simulink model "physical_lab5_bandwidth"  (R2024b)
settings: Solver=ode15s  StartTime=0.0  StopTime=0.0001  MaxStep=1.6666666666666667e-08  RelTol=1e-7  AbsTol=1e-9
model workspace (MAT data in the model file):
  physical_input = timeseries
  physical_input.Name = 'unnamed'
  physical_input.DataInfo = tsdata.datametadata
  physical_input.DataInfo.Interpolation = tsdata.interpolation
  physical_input.DataInfo.Interpolation.Fhandle : function handle (value not decoded)
  physical_input.DataInfo.Interpolation.Name = 'linear'
  physical_input.TimeInfo = tsdata.timemetadata
  physical_input.TimeInfo.Length = 6001
  physical_input.TimeInfo.DuplicateTimes = 0
  physical_input.TimeInfo.Time_ = [0 1.66666666667e-08 3.33333333333e-08 5e-08 6.66666666667e-08 8.33333333333e-08 1e-07 1.16666666667e-07 1.33333333333e-07 1.5e-07 1.66666666667e-07 1.83333333333e-07 ... (6001 elements, 6001x1)]
  physical_input.TimeInfo.Initialized = 1
  physical_input.QualityInfo = tsdata.qualmetadata
  physical_input.Data_ = [0 0.000523589205812 0.00104712099417 0.00157053795391 0.00209378268646 0.00261679781215 0.00313952597647 0.00366190985638 0.00418389216662 0.00470541566593 0.00522642316338 0.00574685752464 ... (6001 elements, 6001x1)]
libraries: fl_lib x13, nesl_utility x7
settings Model: Creator=33657  LastModifiedBy=33657

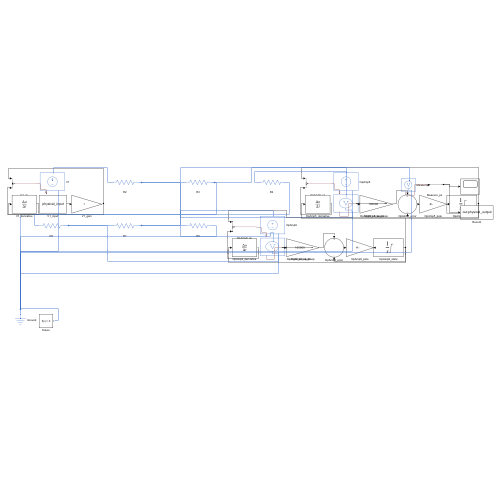
[thumbnail: Simulink's stored preview of the top-level diagram]
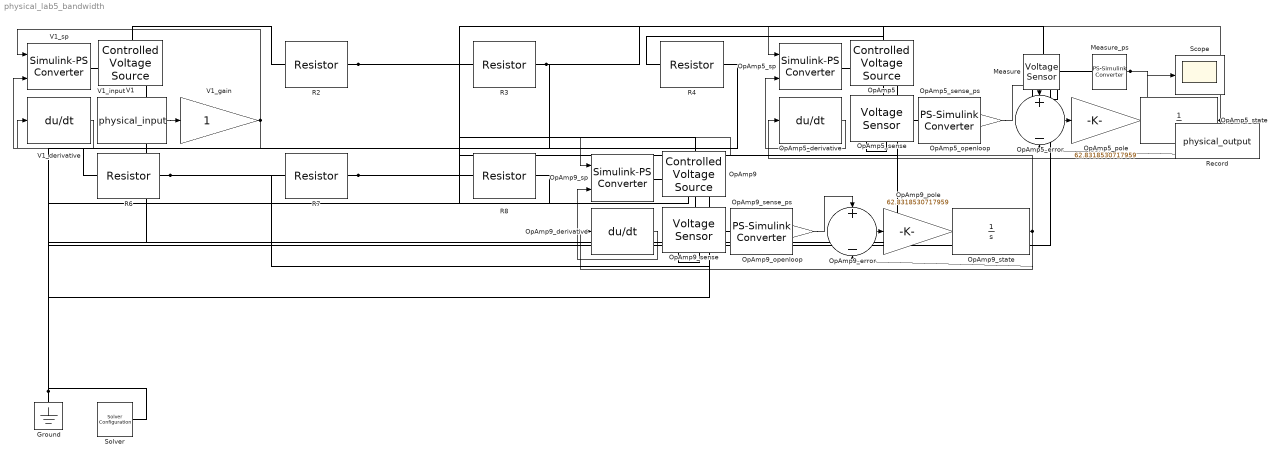
== system physical_lab5_bandwidth ==
  Ground : fl_lib/Electrical/Electrical Elements/Electrical Reference
  Measure : fl_lib/Electrical/Electrical Sensors/Voltage Sensor
  Measure_ps : nesl_utility/PS-Simulink Converter  PhysicalDomain=network_engine_domain  SubClassName=ps_output  LeftPortType=input  RightPortType=output  PseudoPeriodic=off  Frequencies=[]  VectorFormat=inherit  Unit=V  AffineConversion=off
  OpAmp5 : fl_lib/Electrical/Electrical Sources/Controlled Voltage Source
  OpAmp5_derivative : Derivative
  OpAmp5_error : Sum  Inputs=+-
  OpAmp5_openloop : Gain  Gain=100000
  OpAmp5_pole : Gain  Gain=62.8318530717959
  OpAmp5_sense : fl_lib/Electrical/Electrical Sensors/Voltage Sensor
  OpAmp5_sense_ps : nesl_utility/PS-Simulink Converter  PhysicalDomain=network_engine_domain  SubClassName=ps_output  LeftPortType=input  RightPortType=output  PseudoPeriodic=off  Frequencies=[]  VectorFormat=inherit  Unit=V  AffineConversion=off
  OpAmp5_sp : nesl_utility/Simulink-PS Converter  PhysicalDomain=network_engine_domain  SubClassName=ps_input  LeftPortType=input  RightPortType=output  PseudoPeriodic=off  Frequencies=[]  NoiseDistribution=none  NoiseParameters=[]  Unit=V  AffineConversion=off  FilteringAndDerivatives=provide  SimscapeFilterOrder=1  InputFilterTimeConstant=0.001  UdotUserProvided=1
  OpAmp5_state : Integrator  LimitOutput=on  UpperSaturationLimit=15  LowerSaturationLimit=-15
  OpAmp9 : fl_lib/Electrical/Electrical Sources/Controlled Voltage Source
  OpAmp9_derivative : Derivative
  OpAmp9_error : Sum  Inputs=+-
  OpAmp9_openloop : Gain  Gain=100000
  OpAmp9_pole : Gain  Gain=62.8318530717959
  OpAmp9_sense : fl_lib/Electrical/Electrical Sensors/Voltage Sensor
  OpAmp9_sense_ps : nesl_utility/PS-Simulink Converter  PhysicalDomain=network_engine_domain  SubClassName=ps_output  LeftPortType=input  RightPortType=output  PseudoPeriodic=off  Frequencies=[]  VectorFormat=inherit  Unit=V  AffineConversion=off
  OpAmp9_sp : nesl_utility/Simulink-PS Converter  PhysicalDomain=network_engine_domain  SubClassName=ps_input  LeftPortType=input  RightPortType=output  PseudoPeriodic=off  Frequencies=[]  NoiseDistribution=none  NoiseParameters=[]  Unit=V  AffineConversion=off  FilteringAndDerivatives=provide  SimscapeFilterOrder=1  InputFilterTimeConstant=0.001  UdotUserProvided=1
  OpAmp9_state : Integrator  LimitOutput=on  UpperSaturationLimit=15  LowerSaturationLimit=-15
  R{2..4,6..8} (6 alike) : fl_lib/Electrical/Electrical Elements/Resistor  R=100000 Ohm  i_specify=off  i_priority=None  i=0 A  i_nominal_specify=off  i_nominal_value=1  i_nominal_unit=A  v_specify=off  v_priority=None  v=0 V  v_nominal_specify=off  v_nominal_value=1  v_nominal_unit=V
  Record : ToWorkspace  VariableName=physical_output  SaveFormat=Timeseries  SampleTime=-1
  Scope : Scope
  Solver : nesl_utility/Solver Configuration  PhysicalDomain=network_engine_domain  SubClassName=solver  LeftPortType=input  RightPortType=generic  Tones=[]  Harmonics=[]  SimulateNoise=off  Profile=off  UseLocalSampling=off  EnableSwitchedLinearOptims=on  FrequencyDomain=off  UseCCode=off  RelTol=0.001  AbsTol=0.001  MinStep=1e-09  ToWorkspace=off  RevertToSquareIcSolve=off  NumHomotopyIterations=100  PhasorMode=off  PhasorModeNumHarmonics=1  ConsistencySolver=NEWTON_XTOL_AFTER_FTOL  IndexReductionMethod=DerivativeReplacement  DoDC=off  ResidualTolerance=1e-09  ConsistencyTolSource=GLOBAL  ConsistencyAbsTol=0.001  ConsistencyRelTol=0.001  ConsistencyTolFactor=0.001  UseLocalSolver=off  LocalSolverChoice=NE_BACKWARD_EULER_ADVANCER  ResolveIndetEquations=on  FunctionEvalNumThread=1  LocalSolverSampleTime=0.001  DoFixedCost=off  MaxNonlinIter=3  MaxModeIter=2  ComputeImpulses=off  ImpulseIterations=2  LinearAlgebra=auto  LinearAlgebraNumThread=0  EquationFormulation=NE_TIME_EF  DelaysMemoryBudget=1024  AutomaticFiltering=on  FilteringTimeConstant=0.001  PartitionStorageMethod=AS_NEEDED  PartitionMemoryBudget=1024  PartitionMethod=ROBUST  MultibodyUseLocalSolver=off  MultibodyLocalSolverChoice=ODE1  MultibodyLocalSolverSampleTime=0.001
  V1 : fl_lib/Electrical/Electrical Sources/Controlled Voltage Source
  V1_derivative : Derivative
  V1_gain : Gain
  V1_input : FromWorkspace  VariableName=physical_input
  V1_sp : nesl_utility/Simulink-PS Converter  PhysicalDomain=network_engine_domain  SubClassName=ps_input  LeftPortType=input  RightPortType=output  PseudoPeriodic=off  Frequencies=[]  NoiseDistribution=none  NoiseParameters=[]  Unit=V  AffineConversion=off  FilteringAndDerivatives=provide  SimscapeFilterOrder=1  InputFilterTimeConstant=0.001  UdotUserProvided=1
  wires:
  V1_input/1 -> V1_gain/1
  V1_gain/1 -> V1_derivative/1, V1_sp/1
  V1_derivative/1 -> V1_sp/2
  OpAmp5_sense_ps/1 -> OpAmp5_openloop/1
  OpAmp5_openloop/1 -> OpAmp5_error/1
  OpAmp5_error/1 -> OpAmp5_pole/1
  OpAmp5_pole/1 -> OpAmp5_state/1
  OpAmp5_state/1 -> OpAmp5_error/2, OpAmp5_derivative/1, OpAmp5_sp/1
  OpAmp5_derivative/1 -> OpAmp5_sp/2
  OpAmp9_sense_ps/1 -> OpAmp9_openloop/1
  OpAmp9_openloop/1 -> OpAmp9_error/1
  OpAmp9_error/1 -> OpAmp9_pole/1
  OpAmp9_pole/1 -> OpAmp9_state/1
  OpAmp9_state/1 -> OpAmp9_error/2, OpAmp9_derivative/1, OpAmp9_sp/1
  OpAmp9_derivative/1 -> OpAmp9_sp/2
  Measure_ps/1 -> Scope/1, Record/1
  connections:
  Solver/RConn1 -- Ground/LConn1 -- V1/RConn2 -- R4/RConn1 -- OpAmp5/RConn2 -- R8/RConn1 -- OpAmp9/RConn2 -- Measure/RConn2
  V1_sp/RConn1 -- V1/RConn1
  V1/LConn1 -- R2/LConn1
  R3/LConn1 -- R2/RConn1 -- OpAmp5_sense/RConn2
  R4/LConn1 -- OpAmp5_sense/LConn1
  OpAmp5_sense/RConn1 -- OpAmp5_sense_ps/LConn1
  OpAmp5/LConn1 -- R3/RConn1 -- R6/LConn1
  OpAmp5_sp/RConn1 -- OpAmp5/RConn1
  R7/LConn1 -- R6/RConn1 -- OpAmp9_sense/RConn2
  R8/LConn1 -- OpAmp9_sense/LConn1
  OpAmp9_sense/RConn1 -- OpAmp9_sense_ps/LConn1
  OpAmp9/LConn1 -- R7/RConn1 -- Measure/LConn1
  OpAmp9_sp/RConn1 -- OpAmp9/RConn1
  Measure/RConn1 -- Measure_ps/LConn1
